simulink subsystem "DcDcConverterElec_refsub"  (R2023a)
settings: Solver=VariableStepAuto  StartTime=0.0  StopTime=10.0  RelTol=1e-3
undefined symbols (not defined in the file): Minus, Plus
libraries: fl_lib x9, nesl_utility x6, ee_lib x1
settings Model: Creator=isaacito  LastModifiedBy=isaacito
settings SolverCC: AlgebraicLoopSolver=TrustRegion
settings OptimizationCC: ReuseModelBlockBuffer=off
settings DebuggingCC: UnconnectedInputMsg=warning  UnconnectedOutputMsg=warning  UnconnectedLineMsg=warning
settings ModelReferenceCC: EnableRefExpFcnMdlSchedulingChecks=on
settings RTWCC: DLArmComputeVersion=19.05

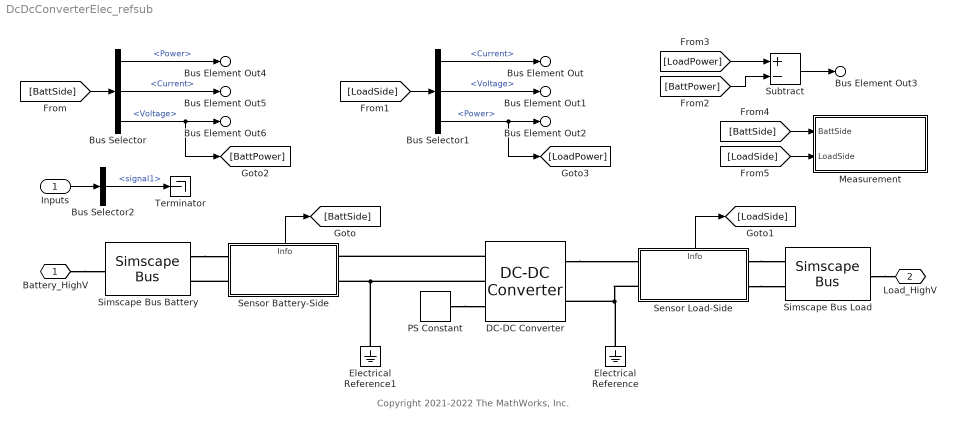
== system DcDcConverterElec_refsub ==
  note: Copyright 2021-2022 The MathWorks, Inc.
  Inputs : Inport
  Bus Selector : BusSelector  OutputSignals=Power,Current,Voltage
  Bus Selector1 : BusSelector  OutputSignals=Current,Voltage,Power
  Bus Selector2 : BusSelector  OutputSignals=signal1
  DC-DC Converter : ee_lib/Semiconductors & Converters/Converters/DC-DC Converter  Vref_option=ee.enum.converters.voltageref.external  v_ref=10 V  P_rated=dcDcConverter.outputPower_kW kW  droop_enabled=false  droop_param=ee.enum.converters.droop.value  droop=0 V/A  droop_percent=0  Vref_droop=10 V  reversible=ee.enum.converters.directionality.bidirectional  G_diode=1e-8 1/Ohm  P_fixed=dcDcConverter.fixedLoss_W W  losses_option=ee.enum.converters.lossesOption.proportionalToSquaredCurrent  eff_rated=dcDcConverter.efficiency_pct  tableOption=ee.enum.converters.lossTableOption.current  i_eff_vec=[1, 2, 3, 4] A  v_eff_vec=[15, 30, 45] V  eff_vec=[90, 80, 70, 60]  eff_2D_table=[90, 85, 80; 80, 75, 70; 70, 65, 60; 60, 55, 50]  model_dynamics=ee.enum.converters.dynamics.no  tau=0.02 s  v_ini=10 V  v1_min=1 V  R1=1000 Ohm  R2=1000 Ohm  enable_fault=ee.enum.faults.faultEnable.no  fault_condition=ee.enum.faults.faultInputCondition.greaterThan  fault_threshold=0.5  T_eff_vec=[280, 300, 320] K  eff_3D_table=repmat([66; 76; 80; 74], 1, 3, 3)  thermal_mass=100 J/K  initial_temperature=298.15 K
      settings: InternalSimscapePortConfiguration="{\"Bottom\":[],\"Left\":[{\"id\":\"p1\",\"label\":\"1+\",\"type\":\"foundation.electrical.electrical\"},{\"id\":\"n1\",\"label\":\"1-\",\"type\":\"foundation.electrical.electrical\"},{\"id\":\"Vref\",\"label\":\"Vref\",\"type\":\"input\"}],\"Right\":[{\"id\":\"p2\",\"label\":\"2+\",\"type\":\"foundation.electrical.electrical\"},{\"id\":\"n2\",\"label\":\"2-\",\"type\":\"foundation.electrical.electrical\"}],\"Top\":[]}"
  Electrical Reference : fl_lib/Electrical/Electrical Elements/Electrical Reference
  Electrical Reference1 : fl_lib/Electrical/Electrical Elements/Electrical Reference
  Measurement : Subsystem
  PS Constant : fl_lib/Physical Signals/Sources/PS Constant  constant=dcDcConverter.outputVoltageRef_V V
  Sensor Battery-Side : Subsystem
      settings: PortSchema="{\"entries\":[{\"content\":{\"sides\":[{\"content\":{\"connectorIds\":[\"LConn1\",\"LConn2\"]},\"type\":\"ConnectorPlacement.EquallySpacedRectSide\",\"uuid\":\"30a3c46a-b3e0-427d-a0c9-e296da4172be\"},{\"content\":{\"connectorIds\":[\"RConn1\",\"RConn2\"],\"side\":\"RIGHT\"},\"type\":\"ConnectorPlacement.EquallySpacedRectSide\",\"uuid\":\"48782190-a487-49f7-9f54-e3a703410830\"},{\"content\":{\"connectorIds\":[\"Out1\"],\"side\":\"TOP\"},\"type\":\"ConnectorPlacement.EquallySpacedRectSide\",\"uuid\":\"37a901e6-af8d-4d93-a097-cadde85f702b\"},{\"content\":{\"connectorIds\":[],\"side\":\"HIDDEN\"},\"type\":\"ConnectorPlacement.EquallySpacedRectSide\",\"uuid\":\"e05a31e4-ac96-47b1-b0f8-1d500f120ecd\"}]},\"type\":\"ConnectorPlacement.EquallySpacedConnector\",\"uuid\":\"392c062c-c64b-4158-94e7-7a4212c653a5\"}],\"packageUris\":[\"http://schema.mathworks.com/mf0/Connector/R2020b\"],\"version\":\"1.0\"}"
  Sensor Load-Side : Subsystem
      settings: PortSchema="{\"entries\":[{\"content\":{\"sides\":[{\"content\":{\"connectorIds\":[\"LConn1\",\"LConn2\"]},\"type\":\"ConnectorPlacement.EquallySpacedRectSide\",\"uuid\":\"30a3c46a-b3e0-427d-a0c9-e296da4172be\"},{\"content\":{\"connectorIds\":[\"RConn1\",\"RConn2\"],\"side\":\"RIGHT\"},\"type\":\"ConnectorPlacement.EquallySpacedRectSide\",\"uuid\":\"48782190-a487-49f7-9f54-e3a703410830\"},{\"content\":{\"connectorIds\":[\"Out1\"],\"side\":\"TOP\"},\"type\":\"ConnectorPlacement.EquallySpacedRectSide\",\"uuid\":\"37a901e6-af8d-4d93-a097-cadde85f702b\"},{\"content\":{\"connectorIds\":[],\"side\":\"HIDDEN\"},\"type\":\"ConnectorPlacement.EquallySpacedRectSide\",\"uuid\":\"e05a31e4-ac96-47b1-b0f8-1d500f120ecd\"}]},\"type\":\"ConnectorPlacement.EquallySpacedConnector\",\"uuid\":\"392c062c-c64b-4158-94e7-7a4212c653a5\"}],\"packageUris\":[\"http://schema.mathworks.com/mf0/Connector/R2020b\"],\"version\":\"1.0\"}"
  Simscape Bus Battery : SimscapeBus  HierarchyStrings=Plus;Minus  ConnectionType=Bus: Bus_HighVoltage
      settings: AttributesFormatString=%<ConnectionType>
  Simscape Bus Load : SimscapeBus  HierarchyStrings=Plus;Minus  ConnectionType=Bus: Bus_HighVoltage
      settings: AttributesFormatString=%<ConnectionType>
  Subtract : Sum  Inputs=+-
  Terminator : Terminator
  Battery_HighV : PMIOPort  Side=Left
  Load_HighV : PMIOPort  Port=2  Side=Right
  Bus Element Out : Outport  PortName=Info  Element=LoadCurr
  Bus Element Out1 : Outport  PortName=Info  Element=LoadV
  Bus Element Out2 : Outport  PortName=Info  Element=LoadPower
  Bus Element Out3 : Outport  PortName=Info  Element=PowerDiff
  Bus Element Out4 : Outport  PortName=Info  Element=BattPower
  Bus Element Out5 : Outport  PortName=Info  Element=BattCurr
  Bus Element Out6 : Outport  PortName=Info  Element=BattV
  wires:
  Sensor Battery-Side/1(Info) -> [BattSide]
  Sensor Load-Side/1(Info) -> [LoadSide]
  [BattSide] -> Bus Selector/1
  [LoadSide] -> Bus Selector1/1
  Bus Selector1/1 -> Bus Element Out/1  "<Current>"
  Bus Selector1/2 -> Bus Element Out1/1  "<Voltage>"
  Bus Selector1/3 -> Bus Element Out2/1, [LoadPower]  "<Power>"
  Bus Selector/1 -> Bus Element Out4/1  "<Power>"
  Bus Selector/2 -> Bus Element Out5/1  "<Current>"
  Bus Selector/3 -> Bus Element Out6/1, [BattPower]  "<Voltage>"
  Subtract/1 -> Bus Element Out3/1
  [BattPower] -> Subtract/2
  [LoadPower] -> Subtract/1
  [BattSide] -> Measurement/1(BattSide)
  [LoadSide] -> Measurement/2(LoadSide)
  Inputs/1 -> Bus Selector2/1
  Bus Selector2/1 -> Terminator/1  "<signal1>"
  connections:
  Electrical Reference/LConn1 -- Sensor Load-Side/LConn2 -- DC-DC Converter/RConn2
  DC-DC Converter/LConn2 -- Electrical Reference1/LConn1 -- Sensor Battery-Side/RConn2
  Battery_HighV/RConn1 -- Simscape Bus Battery/RConn1
  Simscape Bus Load/RConn1 -- Load_HighV/RConn1
  Simscape Bus Battery/LConn1 -- Sensor Battery-Side/LConn1
  Sensor Battery-Side/LConn2 -- Simscape Bus Battery/LConn2
  Sensor Load-Side/RConn1 -- Simscape Bus Load/LConn1
  Sensor Load-Side/RConn2 -- Simscape Bus Load/LConn2
  DC-DC Converter/RConn1 -- Sensor Load-Side/LConn1
  DC-DC Converter/LConn1 -- Sensor Battery-Side/RConn1
  PS Constant/RConn1 -- DC-DC Converter/LConn3

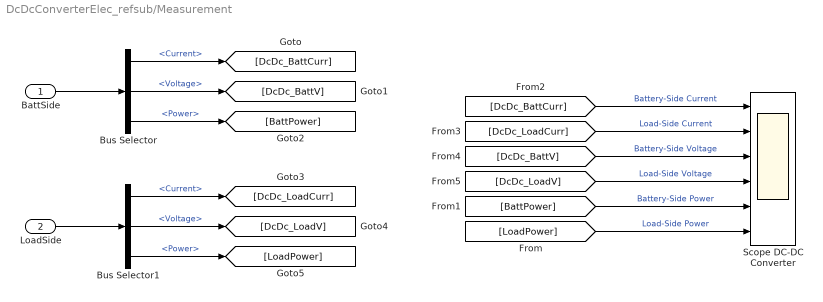
== system DcDcConverterElec_refsub/Measurement ==
  BattSide : Inport
  LoadSide : Inport  Port=2
  Bus Selector : BusSelector  OutputSignals=Current,Voltage,Power
  Bus Selector1 : BusSelector  OutputSignals=Current,Voltage,Power
  Scope DC-DC Converter : Scope  NumInputPorts=6
  wires:
  [LoadPower] -> Scope DC-DC Converter/6  "Load-Side Power"
  [BattPower] -> Scope DC-DC Converter/5  "Battery-Side Power"
  [DcDc_LoadV] -> Scope DC-DC Converter/4  "Load-Side Voltage"
  [DcDc_BattV] -> Scope DC-DC Converter/3  "Battery-Side Voltage"
  [DcDc_LoadCurr] -> Scope DC-DC Converter/2  "Load-Side Current"
  [DcDc_BattCurr] -> Scope DC-DC Converter/1  "Battery-Side Current"
  Bus Selector1/3 -> [LoadPower]  "<Power>"
  Bus Selector1/2 -> [DcDc_LoadV]  "<Voltage>"
  Bus Selector1/1 -> [DcDc_LoadCurr]  "<Current>"
  LoadSide/1 -> Bus Selector1/1
  Bus Selector/3 -> [BattPower]  "<Power>"
  Bus Selector/2 -> [DcDc_BattV]  "<Voltage>"
  Bus Selector/1 -> [DcDc_BattCurr]  "<Current>"
  BattSide/1 -> Bus Selector/1

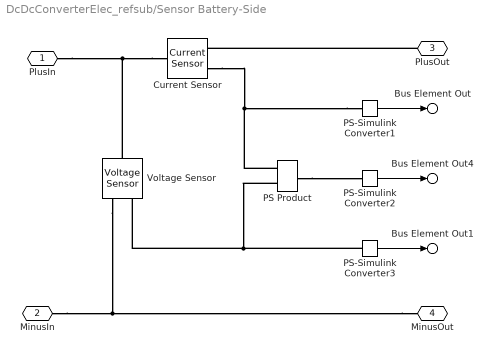
== system DcDcConverterElec_refsub/Sensor Battery-Side ==
  Current Sensor : fl_lib/Electrical/Electrical Sensors/Current Sensor
  PS Product : fl_lib/Physical Signals/Functions/PS Product
  PS-Simulink Converter1 : nesl_utility/PS-Simulink Converter  PhysicalDomain=network_engine_domain  SubClassName=ps_output  LeftPortType=input  RightPortType=output  PseudoPeriodic=off  Frequencies=[]  VectorFormat=1-D array  Unit=A  AffineConversion=off
  PS-Simulink Converter2 : nesl_utility/PS-Simulink Converter  PhysicalDomain=network_engine_domain  SubClassName=ps_output  LeftPortType=input  RightPortType=output  PseudoPeriodic=off  Frequencies=[]  VectorFormat=1-D array  Unit=kW  AffineConversion=off
  PS-Simulink Converter3 : nesl_utility/PS-Simulink Converter  PhysicalDomain=network_engine_domain  SubClassName=ps_output  LeftPortType=input  RightPortType=output  PseudoPeriodic=off  Frequencies=[]  VectorFormat=1-D array  Unit=V  AffineConversion=off
  Voltage Sensor : fl_lib/Electrical/Electrical Sensors/Voltage Sensor
  PlusIn : PMIOPort  Side=Left
  MinusIn : PMIOPort  Port=2  Side=Left
  PlusOut : PMIOPort  Port=3  Side=Right
  MinusOut : PMIOPort  Port=4  Side=Right
  Bus Element Out : Outport  PortName=Info  Element=Current
  Bus Element Out1 : Outport  PortName=Info  Element=Voltage
  Bus Element Out4 : Outport  PortName=Info  Element=Power
  wires:
  PS-Simulink Converter1/1 -> Bus Element Out/1
  PS-Simulink Converter3/1 -> Bus Element Out1/1
  PS-Simulink Converter2/1 -> Bus Element Out4/1
  connections:
  PS-Simulink Converter1/LConn1 -- PS Product/LConn1 -- Current Sensor/RConn1
  MinusOut/RConn1 -- Voltage Sensor/RConn2 -- MinusIn/RConn1
  Current Sensor/LConn1 -- Voltage Sensor/LConn1 -- PlusIn/RConn1
  PlusOut/RConn1 -- Current Sensor/RConn2
  Voltage Sensor/RConn1 -- PS Product/LConn2 -- PS-Simulink Converter3/LConn1
  PS Product/RConn1 -- PS-Simulink Converter2/LConn1

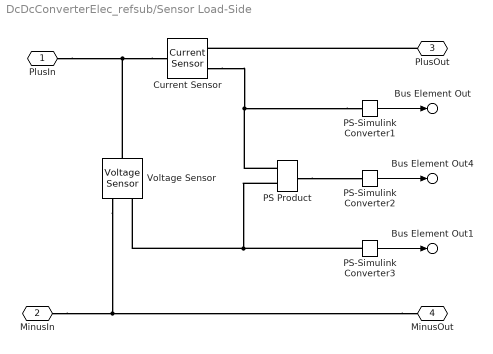
== system DcDcConverterElec_refsub/Sensor Load-Side ==
  Current Sensor : fl_lib/Electrical/Electrical Sensors/Current Sensor
  PS Product : fl_lib/Physical Signals/Functions/PS Product
  PS-Simulink Converter1 : nesl_utility/PS-Simulink Converter  PhysicalDomain=network_engine_domain  SubClassName=ps_output  LeftPortType=input  RightPortType=output  PseudoPeriodic=off  Frequencies=[]  VectorFormat=1-D array  Unit=A  AffineConversion=off
  PS-Simulink Converter2 : nesl_utility/PS-Simulink Converter  PhysicalDomain=network_engine_domain  SubClassName=ps_output  LeftPortType=input  RightPortType=output  PseudoPeriodic=off  Frequencies=[]  VectorFormat=1-D array  Unit=kW  AffineConversion=off
  PS-Simulink Converter3 : nesl_utility/PS-Simulink Converter  PhysicalDomain=network_engine_domain  SubClassName=ps_output  LeftPortType=input  RightPortType=output  PseudoPeriodic=off  Frequencies=[]  VectorFormat=1-D array  Unit=V  AffineConversion=off
  Voltage Sensor : fl_lib/Electrical/Electrical Sensors/Voltage Sensor
  PlusIn : PMIOPort  Side=Left
  MinusIn : PMIOPort  Port=2  Side=Left
  PlusOut : PMIOPort  Port=3  Side=Right
  MinusOut : PMIOPort  Port=4  Side=Right
  Bus Element Out : Outport  PortName=Info  Element=Current
  Bus Element Out1 : Outport  PortName=Info  Element=Voltage
  Bus Element Out4 : Outport  PortName=Info  Element=Power
  wires:
  PS-Simulink Converter1/1 -> Bus Element Out/1
  PS-Simulink Converter3/1 -> Bus Element Out1/1
  PS-Simulink Converter2/1 -> Bus Element Out4/1
  connections:
  PS-Simulink Converter1/LConn1 -- PS Product/LConn1 -- Current Sensor/RConn1
  MinusOut/RConn1 -- Voltage Sensor/RConn2 -- MinusIn/RConn1
  Current Sensor/LConn1 -- Voltage Sensor/LConn1 -- PlusIn/RConn1
  PlusOut/RConn1 -- Current Sensor/RConn2
  Voltage Sensor/RConn1 -- PS Product/LConn2 -- PS-Simulink Converter3/LConn1
  PS Product/RConn1 -- PS-Simulink Converter2/LConn1
